simulink model "PassVeh14DOF"  (R2026b)
settings: Solver=ode23tb  StopTime=inf  FixedStep=.001  RelTol=1e-1  EnableMultiTasking=on
model workspace (MAT data in the model file):
  AlgnTrqCambCompl = [0 0 0 0]
  AlgnTrqSteerCompl = [0 0 0 0]
  AxlIxx = 62.3745166667
  AxlM = 160
  BumpCamber = [0 0 0 0]
  BumpCaster = [0 0 0 0]
  BumpSteer = [0 0 0 0]
  CambVsSteerAng = [0 0 0 0]
  CastVsSteerAng = [0 0 0 0]
  Cps = 2
  Cz = 5565.2246438
  CzWhlAxl = 11490.971257
  DCT_Param : object (value not decoded)
  Downshift_Speeds = [9.5625 12.9375 16.3125 19.6875 23.0625 26.4375 29.8125 33.1875 36.5625 39.9375 43.3125 46.6875 ... (28 elements, 4x7)]
  F0z = [2886 2907]
  F0zWhlAxl = 2907
  Hmax = 0.25
  Kz = 52451.0065793
  KzWhlAxl = 138031.612078
  LatCambCompl = [0 0 0 0]
  LatSteerCompl = [0 0 0 0]
  LatWhlCtrComplLat = [0 0 0 0]
  LatWhlCtrComplLng = [0  0  0  0; 0  0  0  0]
  LatWhlCtrDisp = [0 0 0 0]
  LngCambCompl = [0  0  0  0; 0  0  0  0]
  LngCastCompl = [0  0  0  0; 0  0  0  0]
  LngSteerCompl = [0  0  0  0; 0  0  0  0]
  LngWhlCtrCompl = [0  0  0  0; 0  0  0  0]
  LngWhlCtrDisp = [0 0 0 0]
  MotRatios = [1 1]
  NCyl = 6
  NrmlWhlFrcOff = [2886 2886 2907 2907]
  NrmlWhlRates = [52.4510065793 52.4510065793 52.4510065793 52.4510065793]
  Pedal_Positions = [0.1 0.4 0.5 0.9]
  Pstd = 101325
  Rair = 287
  RollCamber : object (value not decoded)
  RollCaster : object (value not decoded)
  RollSteer : object (value not decoded)
  RollStiffArb = [0 0]
  RollStiffArbFrnt = 800
  RollStiffNoArb = [0 0]
  RollStiffNoArbFrnt = 0
  RollStiffNoTwstRear = 0
  ShckFrcVsCompRate = [5.5652246438 5.5652246438 5.5652246438 5.5652246438]
  StatCamber = [0 0 0 0]
  StatCaster = [0 0 0 0]
  StatLdWhlR = [0.3 0.3 0.3 0.3]
  StatToe = [0 0 0 0]
  Trans : object (value not decoded)
  Tstd = 293.15
  Upshift_Speeds = [12.9375 16.3125 19.6875 33 26.4375 29.8125 33.1875 52.5 39.9375 43.3125 46.6875 77.25 ... (28 elements, 4x7)]
  VEH : object (value not decoded)
  Vd = 0.00346
  VrtLdTrnsfr = [0 0 0 0]
  WH : Mass (value not decoded)
  dt3D = 0.05
  f_air = [0 0 0 0 0 0 0 0 0 0 0 0 ... (256 elements, 16x16)]
  f_co = [0 0 0 0 0 0 0 0 0 0 0 0 ... (256 elements, 16x16)]
  f_co2 = [0 0 0 0 0 0 0 0 0 0 0 0 ... (256 elements, 16x16)]
  f_eff = [352.135682859 352.135682859 320.724378192 303.655312657 295.930136708 291.240087194 291.240271258 291.240312459 291.240275452 291.240198499 291.240100781 291.240018769 ... (256 elements, 16x16)]
  f_fuel = [0 0 0 0 0 0 0 0 0 0 0 0 ... (256 elements, 16x16)]
  f_hc = [0 0 0 0 0 0 0 0 0 0 0 0 ... (256 elements, 16x16)]
  f_nox = [0 0 0 0 0 0 0 0 0 0 0 0 ... (256 elements, 16x16)]
  f_pm = [0 0 0 0 0 0 0 0 0 0 0 0 ... (256 elements, 16x16)]
  f_susp_axl_bp = [1 2]
  f_susp_dz_bp = [-0.325022776267 -0.315022776267 -0.305022776267 -0.205022776267 -0.105022776267 -0.00502277626717 0.0949772237328 0.194977223733 0.204977223733 0.214977223733]
  f_susp_dzdot_bp = [-3 -0.3 -0.2 -0.1 0 0.1 0.2 0.3 3]
  f_susp_fmz = [-144070.391448 -93629.24037 -75929.1118915 -20630.5828179 -15385.48216 -10140.3815021 -4895.28084414 349.819813785 -31916.3973792 18437.6709544 -83996.1993354 -33555.0482577 ... (43920 elements, 10x9x61x2x4)]
  f_susp_geom = [0 0 0 0 0 0 0 0 0 0 0 0 ... (3660 elements, 10x61x2x3)]
  f_susp_strgdelta_bp = [-0.523598775598 -0.506145483078 -0.488692190558 -0.471238898038 -0.453785605519 -0.436332312999 -0.418879020479 -0.401425727959 -0.383972435439 -0.366519142919 -0.349065850399 -0.331612557879 ... (61 elements, 1x61)]
  f_tbrake = [0 76.8593923996 105.140482948 131.533638111 157.926793274 176.658631717 176.65727296 176.656856686 176.656879077 176.657093756 176.657404516 176.65772406 ... (256 elements, 16x16)]
  f_tbrake_n_bpt = [0 649.519052838 912.419621844 1175.32019085 1438.22075986 1701.12132886 1964.02189787 2226.92246687 2489.82303588 2752.72360489 3015.62417389 3278.5247429 ... (16 elements, 1x16)]
  f_tbrake_t_bpt = [0 34.6410161514 61.0341713143 87.4273264773 113.82048164 140.213636803 166.606791966 192.999947129 219.393102292 245.786257455 272.179412618 298.572567781 ... (16 elements, 1x16)]
  f_texh = [766.752464599 766.752464599 786.17542386 801.679939032 884.591982581 910.574397722 910.571871054 910.570774534 910.570601632 910.570821151 910.571247242 910.571639815 ... (256 elements, 16x16)]
  f_twc_eff_co = [0.17 0.25 0.45 0.99 0.99 0.99 0.99]
  f_twc_eff_hc = [0.21 0.375 0.75 0.98 0.98 0.98 0.98]
  f_twc_eff_lam = [0.909090909 0.944055944 0.979020979 1 1.013986014 1.048951049 1.083916084]
  f_twc_eff_nox = [0.98 0.98 0.98 0.97 0.05 0.02 0]
  numWheel = 4
symbols that are objects in the model workspace (value not decoded): VEH
libraries: vehdynlibtire x12, vehdynlibsuspension x8, autolibutils x5, sharedtransform x5, shared6dof x2, vehdynlibeom x1, vehdynlibtirecommon x1, matrix_library x1
(part 2 of 9)

== system PassVeh14DOF/Suspension ==
  Steering : Inport
  Vehicle : Inport  Port=2
  Wheel : Inport  Port=3
  Double Wishbone Suspension : Subsystem  VariantControl=1
      mask Display: image('suspdw.png');
  Independent Mapped Front Suspension Mapped Solid Axle Rear Suspension : Subsystem  VariantControl=2
      mask Display: image([imread('suspindmap.png');imread('suspsamap.png')]);
  Kinematics and Compliance Independent Suspension : Subsystem  VariantControl=6
      mask Display: image('suspkandc.png');
  MacPherson Front Suspension Solid Axle Rear Suspension : Subsystem  VariantControl=3
      mask Display: image([imread('suspmacp.png');imread('suspsacoil.png')]);
  MacPherson Suspension : Subsystem  VariantControl=4
      mask Display: image('suspmacp.png');
  Mapped Suspension : Subsystem  VariantControl=5
      mask Display: image('suspindmap.png');
  Suspension : Outport  VectorParamsAs1DForOutWhenUnconnected=off

== system PassVeh14DOF/Vehicle ==
  Suspension : Inport
  Wind : Inport  Port=2
  Constant1 : Constant  Value=[0;0;0]
  Suspension to Chasiss Transforms : Subsystem
  Terminator{,1..5} (6 alike) : Terminator
  Vehicle Body 6DOF : vehdynlibeom/Vehicle Body 6DOF  extPos=on  extVel=on  extEuler=on  extRotRate=on  htchFMode=off  htchMMode=off  m=VEH.Mass  a=VEH.FrontAxlePositionfromCG  b=VEH.RearAxlePositionfromCG  d=0  h=VEH.HeightCG  dh=1  hl=0  hh=0.1  Xe_o=[VEH.InitialLongPosition,VEH.InitialLatPosition,VEH.InitialVertPosition]  xbdot_o=[VEH.InitialLongVel,VEH.InitialLatVel,VEH.InitialVertVel]  eul_o=[VEH.InitialRollAngle,VEH.InitialPitchAngle,VEH.InitialYawAngle]  p_o=[VEH.InitialRollRate,VEH.InitialPitchRate,VEH.InitialYawRate]  Iveh=[VEH.RollMomentInertia 0 0; 0 VEH.PitchMomentInertia 0; 0 0 VEH.YawMomentInertia]  w=VEH.TrackWidth.*[1 1]  z1m=0  z1R=[-.25,.125,.15]  z1I=[1.4,-.2,.1;-.2,1.4,.1;.1,.1,2.25].*0  z2m=0  z2R=[1.4,0,.8]  z2I=[1.4,-.2,.1;-.2,1.4,.1;.1,.1,2.25].*0  z3m=0  z3R=[.75,-.5,.4]  z3I=[5,-.1,-2;-2,9,.1;-.1,.1,6].*0  z4m=0  z4R=[.75,.5,.4]  z4I=[5,-.1,-2;-2,9,.1;-.1,.1,6].*0  z5m=0  z5R=[1.25,-.5,.4]  z5I=[5,-.1,-2;-2,9,.1;-.1,.1,6].*0  z6m=0  z6R=[1.25,-.5,.4]  z6I=[5,-.1,-2;-2,9,.1;-.1,.1,6].*0  z7m=0  z7R=[2,0,.25]  z7I=[1.4,-.2,.1;-.2,1.4,.1;.1,.1,2.25].*0  Af=VEH.FrontalArea  Cd=.3  Cl=.1  Cpm=.1  beta_w=[0,0.1745,0.3491,0.5236,0.6981,0.8727,1.0472,1.2217,1.3963,1.5708]  Cs=[0.1000,0.1000,0.1000,0.1000,0.1000,0.1000,0.1000,0.1000,0.1000,0.1000]  Cym=[0,0,0.0667,0.1000,0.1333,0.1667,0.2000,0.2333,0.2667,0.3000]  Pabs=101325  extTamb=off  Tair=273  g=9.81  xdot_tol=.1  longOff=0  latOff=0  vertOff=0.0112  wrapAng=off  aMode=2
  VehFdbk : Outport  VectorParamsAs1DForOutWhenUnconnected=off
  wires:
  Vehicle Body 6DOF/1 -> VehFdbk/1, Suspension to Chasiss Transforms/1(VehFdbk)  "VehFdbk"
  Vehicle Body 6DOF/7 -> Terminator5/1
  Constant1/1 -> Vehicle Body 6DOF/4
  Wind/1 -> Vehicle Body 6DOF/5
  Vehicle Body 6DOF/2 -> Terminator/1
  Suspension/1 -> Suspension to Chasiss Transforms/2(Suspension)
  Suspension to Chasiss Transforms/1(FsB) -> Vehicle Body 6DOF/1
  Suspension to Chasiss Transforms/3(Fext) -> Vehicle Body 6DOF/3
  Vehicle Body 6DOF/5 -> Terminator3/1
  Vehicle Body 6DOF/6 -> Terminator4/1
  Vehicle Body 6DOF/3 -> Terminator1/1
  Vehicle Body 6DOF/4 -> Terminator2/1
  Suspension to Chasiss Transforms/2(MsB) -> Vehicle Body 6DOF/2

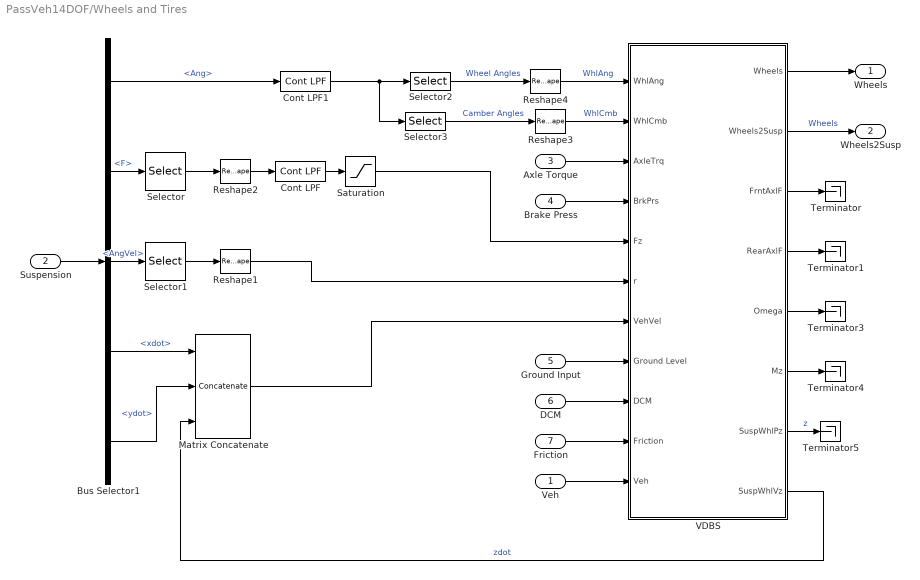
== system PassVeh14DOF/Wheels and Tires ==
  Veh : Inport
  Suspension : Inport  Port=2
  Axle Torque : Inport  Port=3
  Brake Press : Inport  Port=4  Unit=Pa
  Ground Input : Inport  Port=5
  DCM : Inport  Port=6
  Friction : Inport  Port=7  PortDimensions=4
  Bus Selector1 : BusSelector  OutputSignals=Whl.Ang,Whl.F,Whl.AngVel,Whl.xdot,Whl.ydot
  Cont LPF : autolibutils/Cont LPF  wc=100*2*pi  AbsoluteTolerance=auto  aMode=2
  Cont LPF1 : autolibutils/Cont LPF  wc=100*2*pi  AbsoluteTolerance=1e-2  aMode=2
  Matrix Concatenate : Concatenate  NumInputs=3  Mode=Multidimensional array
  Reshape{1..4} (4 alike) : Reshape
  Saturation : Saturate  UpperLimit=inf  LowerLimit=-10*9.81*2000  ZeroCross=off
  Selector : Selector  NumberOfDimensions=2  InputPortWidth=3  IndexOptions=Index vector (dialog),Select all  Indices=[3],1  OutputSizes=1,1
  Selector1 : Selector  NumberOfDimensions=2  InputPortWidth=1  IndexOptions=Index vector (dialog),Select all  Indices=[3],1  OutputSizes=1,1
  Selector2 : Selector  NumberOfDimensions=2  InputPortWidth=3  IndexOptions=Index vector (dialog),Select all  Indices=3,1  OutputSizes=1,1
  Selector3 : Selector  NumberOfDimensions=2  InputPortWidth=3  IndexOptions=Index vector (dialog),Select all  Indices=1,1  OutputSizes=1,1
  Terminator{,1,3..5} (5 alike) : Terminator
  VDBS : Subsystem  VariantControl=0
  Wheels : Outport  VectorParamsAs1DForOutWhenUnconnected=off
  Wheels2Susp : Outport  Port=2  VectorParamsAs1DForOutWhenUnconnected=off
  wires:
  Bus Selector1/2 -> Selector/1  "<F>"
  VDBS/3(FrntAxlF) -> Terminator/1
  VDBS/4(RearAxlF) -> Terminator1/1
  VDBS/5(Omega) -> Terminator3/1
  VDBS/6(Mz) -> Terminator4/1
  Selector1/1 -> Reshape1/1
  Matrix Concatenate/1 -> VDBS/7(VehVel)
  Axle Torque/1 -> VDBS/3(AxleTrq)
  Reshape4/1 -> VDBS/1(WhlAng)  "WhlAng"
  Reshape3/1 -> VDBS/2(WhlCmb)  "WhlCmb"
  Selector/1 -> Reshape2/1
  Saturation/1 -> VDBS/5(Fz)
  Ground Input/1 -> VDBS/8(Ground Level)
  VDBS/8(SuspWhlVz) -> Matrix Concatenate/3  "zdot"
  Bus Selector1/1 -> Cont LPF1/1  "<Ang>"
  Selector3/1 -> Reshape3/1  "Camber Angles"
  Suspension/1 -> Bus Selector1/1
  Bus Selector1/4 -> Matrix Concatenate/1  "<xdot>"
  Bus Selector1/5 -> Matrix Concatenate/2  "<ydot>"
  VDBS/7(SuspWhlPz) -> Terminator5/1  "z"
  Reshape2/1 -> Cont LPF/1
  Bus Selector1/3 -> Selector1/1  "<AngVel>"
  Reshape1/1 -> VDBS/6(r)
  Brake Press/1 -> VDBS/4(BrkPrs)
  Friction/1 -> VDBS/10(Friction)
  Cont LPF/1 -> Saturation/1
  Cont LPF1/1 -> Selector3/1, Selector2/1
  Selector2/1 -> Reshape4/1  "Wheel Angles"
  Veh/1 -> VDBS/11(Veh)
  VDBS/2(Wheels2Susp) -> Wheels2Susp/1  "Wheels"
  VDBS/1(Wheels) -> Wheels/1
  DCM/1 -> VDBS/9(DCM)

== system PassVeh14DOF/Suspension/Double Wishbone Suspension ==
  Wheel : Inport
  Steering : Inport  Port=2
  Vehicle : Inport  Port=3
  Bus Creator1 : BusCreator  Inputs=6
  Bus Creator2 : BusCreator  Inputs=2
  Bus Creator3 : BusCreator  Inputs=2
  Bus Creator4 : BusCreator  Inputs=6
  Bus Selector : BusSelector  OutputSignals=z,RL,zdot,Fx,Fy,M
  Bus Selector1 : BusSelector  OutputSignals=P,V
  Bus Selector2 : BusSelector  OutputSignals=SuspFrame.z
  Independent Suspension – Double Wishbone : vehdynlibsuspension/Independent Suspension - Double Wishbone  ActiveDampEn=off  NumAxl=2  NumWhlsByAxl=[2 2]  StrgEnByAxl=[1 0]  AntiSwayEnByAxl=[1 0]  WhlNumVec="[1  2  1  2]"  AxleNumVec="[1  1  2  2]"  SuspTypesByAxle="[1  1]"  SuspImage=suspdw.png  IdealSuspEn=on  IdealSuspAxles="[1  2]"  Kz=Kz  F0z=F0z  Cz=Cz  Hmax=Hmax  f_act_susp_cz=[10000 10000;10000 10000]  f_act_susp_duty_bpt=[0 1]  f_act_susp_zdot_bpt=[-1 1]  Toe=0.  RollStrgSlp=0.  ToeStrgSlp=0.  Caster=0.  CasterHslp=0.  CasterStrgSlp=0.  Camber=0.  CamberHslp=0.  CamberStrgSlp=0.  StrgHgtSlp=0.1432  MappedSuspEn=off  MappedSuspAxles="[1  2]"  f_susp_axl_bp=[1 2]  f_susp_dz_bp=[-0.15 -0.14 -0.13 -0.12 -0.11 -0.10 -0.09 -0.08 -0.07 -0.06 -0.05 -0.04 -0.03 -0.02 -0.01 0.00 0.01 0.02 0.03 0.04 0.05 0.06 0.07 0.08 0.09 0.10 0.11 0.12 0.13 0.14 0.15]  f_susp_dzdot_bp=[-0.15 -0.14 -0.13 -0.12 -0.11 -0.10 -0.09 -0.08 -0.07 -0.06 -0.05 -0.04 -0.03 -0.02 -0.01 0.00 0.01 0.02 0.03 0.04 0.05 0.06 0.07 0.08 0.09 0.10 0.11 0.12 0.13 0.14 0.15]  f_susp_fmz=zeros(31,31,61,2,4)  f_susp_geom=zeros(31,61,2,3)  f_susp_strgdelta_bp=[-30,-29,-28,-27,-26,-25,-24,-23,-22,-21,-20,-19,-18,-17,-16,-15,-14,-13,-12,-11,-10,-9,-8,-7,-6,-5,-4,-3,-2,-1,0,1,2,3,4,5,6,7,8,9,10,11,12,13,14,15,16,17,18,19,20,21,22,23,24,25,26,27,28,29,30]  AntiSwayR=0.2  AntiSwayNtrlAng=0.5236  AntiSwayTrsK=8e2
  Selector1 : Selector  NumberOfDimensions=2  IndexOptions=Index vector (dialog),Select all  Indices=1,1  OutputSizes=1,1
  Selector2 : Selector  NumberOfDimensions=2  IndexOptions=Index vector (dialog),Select all  Indices=2,1  OutputSizes=1,1
  Steer Rate Adapter : Subsystem
  Steering Adapter : Subsystem
  Terminator : Terminator
  Terminator1 : Terminator
  Vehicle Adapter : Subsystem
  Wheel  Adapter : Subsystem
  Wheel1 : InportShadow
  Suspension : Outport  VectorParamsAs1DForOutWhenUnconnected=off
  wires:
  Bus Creator3/1 -> Suspension/1
  Steering Adapter/1(StrgAng) -> Independent Suspension – Double Wishbone/9
  Independent Suspension – Double Wishbone/1 -> Terminator/1
  Wheel  Adapter/6(RL) -> Bus Creator4/6
  Bus Selector1/1 -> Independent Suspension – Double Wishbone/7  "<P>"
  Wheel  Adapter/2(WhlFy) -> Bus Creator4/2  "Fy"
  Wheel/1 -> Wheel  Adapter/1(Wheels)
  Steer Rate Adapter/1(AngVel) -> Bus Creator1/6  "AngVel"
  Bus Creator4/1 -> Bus Selector/1
  Bus Creator2/1 -> Bus Creator3/1  "Veh"
  Vehicle Adapter/2(VehVbody) -> Selector1/1, Selector2/1  "V"
  Selector2/1 -> Bus Creator1/3  "ydot"
  Bus Selector1/2 -> Independent Suspension – Double Wishbone/8  "<V>"
  Independent Suspension – Double Wishbone/2 -> Bus Creator2/1  "F"
  Bus Selector/2 -> Independent Suspension – Double Wishbone/2  "<RL>"
  Wheel  Adapter/5(M) -> Bus Creator4/5  "M"
  Bus Selector/4 -> Independent Suspension – Double Wishbone/4  "<Fx>"
  Independent Suspension – Double Wishbone/4 -> Bus Creator1/1  "F"
  Steering/1 -> Steering Adapter/1(Steer)
  Selector1/1 -> Bus Creator1/2  "xdot"
  Independent Suspension – Double Wishbone/3 -> Bus Creator2/2  "M"
  Vehicle Adapter/1(VehSusp) -> Bus Selector1/1
  Wheel  Adapter/4(zdot) -> Bus Creator4/4
  Vehicle/1 -> Vehicle Adapter/1(Veh), Steer Rate Adapter/1(Veh)
  Bus Selector/6 -> Independent Suspension – Double Wishbone/6  "<M>"
  Bus Selector/5 -> Independent Suspension – Double Wishbone/5  "<Fy>"
  Bus Selector/1 -> Independent Suspension – Double Wishbone/1  "<z>"
  Wheel  Adapter/3(z) -> Bus Creator4/3
  Independent Suspension – Double Wishbone/6 -> Bus Creator1/4  "Ang"
  Bus Creator1/1 -> Bus Creator3/2  "Whl"
  Wheel  Adapter/1(WhlFx) -> Bus Creator4/1  "Fx"
  Bus Selector/3 -> Independent Suspension – Double Wishbone/3  "<zdot>"
  Independent Suspension – Double Wishbone/5 -> Terminator1/1  "V"
  Bus Selector2/1 -> Bus Creator1/5  "<z>"
  Wheel1/1 -> Bus Selector2/1

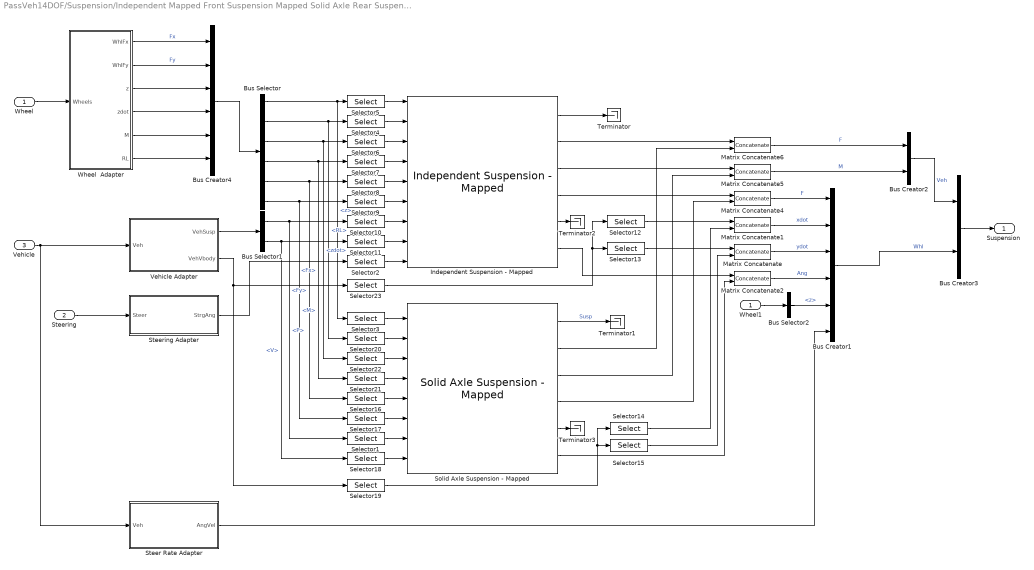
== system PassVeh14DOF/Suspension/Independent Mapped Front Suspension Mapped Solid Axle Rear Suspension ==
  Wheel : Inport
  Steering : Inport  Port=2
  Vehicle : Inport  Port=3
  Bus Creator1 : BusCreator  Inputs=6
  Bus Creator2 : BusCreator  Inputs=2
  Bus Creator3 : BusCreator  Inputs=2
  Bus Creator4 : BusCreator  Inputs=6
  Bus Selector : BusSelector  OutputSignals=z,RL,zdot,Fx,Fy,M
  Bus Selector1 : BusSelector  OutputSignals=P,V
  Bus Selector2 : BusSelector  OutputSignals=SuspFrame.z
  Independent Suspension - Mapped : vehdynlibsuspension/Independent Suspension - Mapped  NumAxl=1  NumWhlsByAxl=2  StrgEnByAxl=1  AntiSwayEnByAxl=1  WhlNumVec="[1  2]"  AxleNumVec="[1  1]"  SuspTypesByAxle=[2]  SuspImage=suspindmap.png  IdealSuspEn=off  IdealSuspAxles="[1  2]"  Kz=64370  F0z=9810  Cz=10000  Hmax=0.5  Toe=2  RollStrgSlp=-13  ToeStrgSlp=0.01  Caster=4  CasterHslp=-13  CasterStrgSlp=0.01  Camber=4  CamberHslp=-13  CamberStrgSlp=0.01  StrgHgtSlp=0.0025  MappedSuspEn=on  MappedSuspAxles=[1]  f_susp_axl_bp=[1 2]  f_susp_dz_bp=f_susp_dz_bp  f_susp_dzdot_bp=f_susp_dzdot_bp  f_susp_fmz=f_susp_fmz  f_susp_geom=f_susp_geom  f_susp_strgdelta_bp=f_susp_strgdelta_bp  NDFLookupOutType=1:4  NDGLookupOutType=1:3  AntiSwayR=0.2  AntiSwayNtrlAng=0.5236  AntiSwayTrsK=8e2
  Matrix Concatenate{,1..2,4..6} (6 alike) : Concatenate  Mode=Multidimensional array  ConcatenateDimension=2
  Selector{1,17..19} (4 alike) : Selector  NumberOfDimensions=2  IndexOptions=Select all,Index vector (dialog)  Indices=[1 2],[3 4]  OutputSizes=1,1
  Selector{9..11,23} (4 alike) : Selector  NumberOfDimensions=2  IndexOptions=Select all,Index vector (dialog)  Indices=[1 2],[1 2]  OutputSizes=1,1
  Selector12 : Selector  NumberOfDimensions=2  InputPortWidth=3  IndexOptions=Index vector (dialog),Select all  Indices=1,1  OutputSizes=1,1
  Selector13 : Selector  NumberOfDimensions=2  InputPortWidth=3  IndexOptions=Index vector (dialog),Select all  Indices=2,1  OutputSizes=1,1
  Selector14 : Selector  NumberOfDimensions=2  InputPortWidth=3  IndexOptions=Index vector (dialog),Select all  Indices=1,1  OutputSizes=1,1
  Selector15 : Selector  NumberOfDimensions=2  InputPortWidth=3  IndexOptions=Index vector (dialog),Select all  Indices=2,1  OutputSizes=1,1
  Selector{3,16,20..22} (5 alike) : Selector  IndexOptions=Index vector (dialog)  Indices=[3 4]  OutputSizes=1
  Selector{2,4..8} (6 alike) : Selector  IndexOptions=Index vector (dialog)  Indices=[1 2]  OutputSizes=1
  Solid Axle Suspension - Mapped : vehdynlibsuspension/Solid Axle Suspension - Mapped  NumAxl=1  NumWhlsByAxl=2  StrgEnByAxl=0  WhlNumVec="[1  2]"  AxleNumVec="[1  1]"  SuspTypesByAxle=[2]  SuspImage=suspsamap.png  AxlIxx=AxlIxx  AxlM=AxlM  TrackCoords=[0 0;VEH.TrackWidth*[-1 1]/2;0 0]  SuspCoords=[0 0;VEH.TrackWidth*[-1 1]/2;0 0]  KzWhlAxl=KzWhlAxl  F0zWhlAxl=F0zWhlAxl  CzWhlAxl=CzWhlAxl  IdealSuspEn=off  IdealSuspAxles="[1  2]"  Kz=64370  F0z=9810  Cz=10000  Hmax=0.5  Toe=2  RollStrgSlp=-13  ToeStrgSlp=0.01  Caster=4  CasterHslp=-13  CasterStrgSlp=0.01  Camber=4  CamberHslp=-13  CamberStrgSlp=0.01  StrgHgtSlp=0.0025  MappedSuspEn=on  MappedSuspAxles=[1]  f_susp_axl_bp=[1 2]  f_susp_dz_bp=f_susp_dz_bp  f_susp_dzdot_bp=f_susp_dzdot_bp  f_susp_fmz=f_susp_fmz  f_susp_geom=f_susp_geom  f_susp_strgdelta_bp=f_susp_strgdelta_bp  NDFLookupOutType=1:4  NDGLookupOutType=1:3
  Steer Rate Adapter : Subsystem
  Steering Adapter : Subsystem
  Terminator{,1..3} (4 alike) : Terminator
  Vehicle Adapter : Subsystem
  Wheel  Adapter : Subsystem
  Wheel1 : InportShadow
  Suspension : Outport  VectorParamsAs1DForOutWhenUnconnected=off
  wires:
  Vehicle Adapter/2(VehVbody) -> Selector19/1, Selector23/1
  Selector22/1 -> Solid Axle Suspension - Mapped/3
  Bus Selector/3 -> Selector22/1, Selector6/1  "<zdot>"
  Solid Axle Suspension - Mapped/4 -> Matrix Concatenate4/2
  Solid Axle Suspension - Mapped/1 -> Terminator1/1  "Susp"
  Selector12/1 -> Matrix Concatenate1/1
  Selector7/1 -> Independent Suspension - Mapped/4
  Selector18/1 -> Solid Axle Suspension - Mapped/8
  Selector13/1 -> Matrix Concatenate/1
  Selector14/1 -> Matrix Concatenate1/2
  Selector21/1 -> Solid Axle Suspension - Mapped/4
  Vehicle/1 -> Vehicle Adapter/1(Veh), Steer Rate Adapter/1(Veh)
  Wheel  Adapter/4(zdot) -> Bus Creator4/4
  Solid Axle Suspension - Mapped/3 -> Matrix Concatenate5/2
  Selector1/1 -> Solid Axle Suspension - Mapped/7
  Matrix Concatenate4/1 -> Bus Creator1/1  "F"
  Selector16/1 -> Solid Axle Suspension - Mapped/5
  Matrix Concatenate5/1 -> Bus Creator2/2  "M"
  Independent Suspension - Mapped/4 -> Matrix Concatenate4/1
  Selector4/1 -> Independent Suspension - Mapped/2
  Selector10/1 -> Independent Suspension - Mapped/7
  Selector9/1 -> Independent Suspension - Mapped/6
  Wheel  Adapter/3(z) -> Bus Creator4/3
  Solid Axle Suspension - Mapped/2 -> Matrix Concatenate6/2
  Wheel/1 -> Wheel  Adapter/1(Wheels)
  Selector5/1 -> Independent Suspension - Mapped/1
  Independent Suspension - Mapped/3 -> Matrix Concatenate5/1
  Selector8/1 -> Independent Suspension - Mapped/5
  Independent Suspension - Mapped/2 -> Matrix Concatenate6/1
  Independent Suspension - Mapped/6 -> Matrix Concatenate2/1
  Selector20/1 -> Solid Axle Suspension - Mapped/2
  Independent Suspension - Mapped/1 -> Terminator/1
  Bus Creator2/1 -> Bus Creator3/1  "Veh"
  Bus Selector/4 -> Selector7/1, Selector21/1  "<Fx>"
  Matrix Concatenate2/1 -> Bus Creator1/4  "Ang"
  Wheel  Adapter/2(WhlFy) -> Bus Creator4/2  "Fy"
  Bus Creator4/1 -> Bus Selector/1
  Selector17/1 -> Solid Axle Suspension - Mapped/6
  Selector2/1 -> Independent Suspension - Mapped/9
  Wheel  Adapter/5(M) -> Bus Creator4/5
  Matrix Concatenate/1 -> Bus Creator1/3  "ydot"
  Steering/1 -> Steering Adapter/1(Steer)
  Matrix Concatenate1/1 -> Bus Creator1/2  "xdot"
  Selector15/1 -> Matrix Concatenate/2
  Selector3/1 -> Solid Axle Suspension - Mapped/1
  Bus Selector1/2 -> Selector11/1, Selector18/1  "<V>"
  Vehicle Adapter/1(VehSusp) -> Bus Selector1/1
  Steering Adapter/1(StrgAng) -> Selector2/1
  Selector6/1 -> Independent Suspension - Mapped/3
  Bus Selector/6 -> Selector9/1, Selector17/1  "<M>"
  Wheel  Adapter/1(WhlFx) -> Bus Creator4/1  "Fx"
  Selector11/1 -> Independent Suspension - Mapped/8
  Wheel  Adapter/6(RL) -> Bus Creator4/6
  Matrix Concatenate6/1 -> Bus Creator2/1  "F"
  Bus Selector1/1 -> Selector10/1, Selector1/1  "<P>"
  Solid Axle Suspension - Mapped/6 -> Matrix Concatenate2/2
  Bus Selector/1 -> Selector3/1, Selector5/1  "<z>"
  Bus Selector/5 -> Selector8/1, Selector16/1  "<Fy>"
  Bus Creator1/1 -> Bus Creator3/2  "Whl"
  Bus Creator3/1 -> Suspension/1
  Bus Selector/2 -> Selector20/1, Selector4/1  "<RL>"
  Steer Rate Adapter/1(AngVel) -> Bus Creator1/6
  Independent Suspension - Mapped/5 -> Terminator2/1
  Solid Axle Suspension - Mapped/5 -> Terminator3/1
  Selector19/1 -> Selector14/1, Selector15/1
  Selector23/1 -> Selector12/1, Selector13/1
  Bus Selector2/1 -> Bus Creator1/5  "<z>"
  Wheel1/1 -> Bus Selector2/1

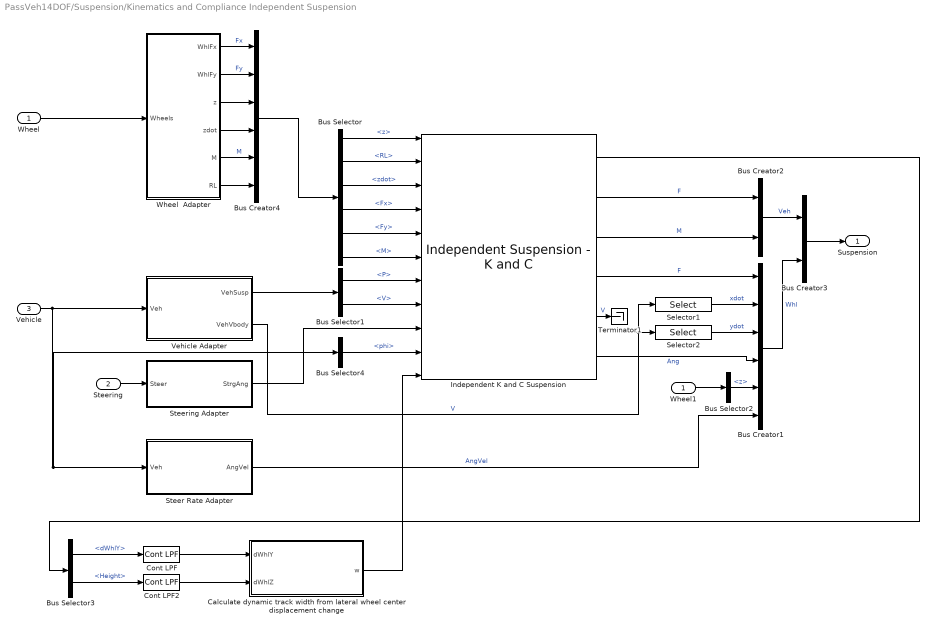
== system PassVeh14DOF/Suspension/Kinematics and Compliance Independent Suspension ==
  Wheel : Inport
  Steering : Inport  Port=2
  Vehicle : Inport  Port=3
  Bus Creator1 : BusCreator  Inputs=6
  Bus Creator2 : BusCreator  Inputs=2
  Bus Creator3 : BusCreator  Inputs=2
  Bus Creator4 : BusCreator  Inputs=6
  Bus Selector : BusSelector  OutputSignals=z,RL,zdot,Fx,Fy,M
  Bus Selector1 : BusSelector  OutputSignals=P,V
  Bus Selector2 : BusSelector  OutputSignals=SuspFrame.z
  Bus Selector3 : BusSelector  OutputSignals=dWhlY,Height
  Bus Selector4 : BusSelector  OutputSignals=InertFrm.Cg.Ang.phi
  Calculate dynamic track width from lateral wheel center displacement change : Subsystem  mask{w=VEH.TrackWidth.*[1 1]}
      mask prompts: w "vdynblks:vehdynVehBody6Dof:blkPrm_w"
      mask DialogControl w Prompt: Track widths [front, rear], w [m]:
  Cont LPF : autolibutils/Cont LPF  wc=100*2*pi  AbsoluteTolerance=auto  aMode=2
  Cont LPF2 : autolibutils/Cont LPF  wc=100*2*pi  AbsoluteTolerance=auto  aMode=2
  Independent K and C Suspension : vehdynlibsuspension/Independent Suspension - K and C  ActiveDampEn=off  NumAxl=2  NumWhlsByAxl=[2 2]  StrgEnByAxl=[1 0]  AntiSwayEnByAxl=[0 0]  WhlNumVec="[1  2  1  2]"  AxleNumVec="[1  1  2  2]"  SuspTypesByAxle="[1  1]"  SuspImage=suspkandc.png  IdealSuspEn=on  IdealSuspAxles="[1  2]"  tanTheta_FL=[0 0 0]  tanTheta_FR=[0 0 0]  tanTheta_RL=[0 0 0]  tanTheta_RR=[0 0 0]  SteerSign=1  LongitudinalSign=1  LateralSign=1  VerticalSign=1  WhlMzSign=1  tanTheta_SVSA_WC_FL=1  tanTheta_SVSA_WC_FR=1  tanTheta_SVSA_WC_RL=1  tanTheta_SVSA_WC_RR=1  tanTheta_SVSA_CP_FL=1  tanTheta_SVSA_CP_FR=1  tanTheta_SVSA_CP_RL=1  tanTheta_SVSA_CP_RR=1  SuspType=Independent front and rear  DrivetrainType=FWD  StrPlusDirection=Right  XPlusDirection=Front  YPlusDirection=Right  ZPlusDirection=Up  WhlMzDirection=Counter-clockwise  ShockType=Constant  ShckFrcVsCompRate=ShckFrcVsCompRate  MotRatios=MotRatios  BumpSteer=BumpSteer  BumpCamber=BumpCamber  BumpCaster=BumpCaster  LatWhlCtrDisp=LatWhlCtrDisp  LngWhlCtrDisp=LngWhlCtrDisp  NrmlWhlRates=NrmlWhlRates  NrmlWhlFrcOff=NrmlWhlFrcOff  RollSteer=RollSteer  RollCamber=RollCamber  RollCaster=RollCaster  RollStiffArb=RollStiffArb  RollStiffNoArb=RollStiffNoArb  RollStiffArbFrnt=RollStiffArbFrnt  RollStiffNoArbFrnt=RollStiffNoArbFrnt  RollStiffNoTwstRear=RollStiffNoTwstRear  CambVsSteerAng=CambVsSteerAng  CastVsSteerAng=CastVsSteerAng  LngSteerCompl=LngSteerCompl  LngCambCompl=LngCambCompl  LngCastCompl=LngCastCompl  LngWhlCtrCompl=LngWhlCtrCompl  LatWhlCtrComplLng=LatWhlCtrComplLng  LatSteerCompl=LatSteerCompl  LatCambCompl=LatCambCompl  LatWhlCtrComplLat=LatWhlCtrComplLat  LatSteerComplOpp=struct('FL',[-2. -1.;0 0;2. 1.],'FR',[-2. 1.;0 0;2. -1.],'RL',[-2. -1.;0 0;2. 1.],'RR',[-2. 1.;0 0;2. -1.])  LatCambComplOpp=struct('FL',[-2. -1.;0 0;2. 1.],'FR',[-2. 1.;0 0;2. -1.],'RL',[-2. -1.;0 0;2. 1.],'RR',[-2. 1.;0 0;2. -1.])  LatWhlCtrComplLatOpp=struct('FL',[-2. -5.;0 0;2. 5.],'FR',[-2. 5.;0 0;2. -5.],'RL',[-2. -5.;0 0;2. 5.],'RR',[-2. 5.;0 0;2. -5.])  AlgnTrqSteerCompl=AlgnTrqSteerCompl  AlgnTrqCambCompl=AlgnTrqCambCompl  VrtLdTrnsfr=VrtLdTrnsfr  LatSteerComplPar=struct('FL',[-2. -1.;0 0;2. 1.],'FR',[-2. 1.;0 0;2. -1.],'RL',[-2. -1.;0 0;2. 1.],'RR',[-2. 1.;0 0;2. -1.])  LatCambComplPar=struct('FL',[-2. -1.;0 0;2. 1.],'FR',[-2. 1.;0 0;2. -1.],'RL',[-2. -1.;0 0;2. 1.],'RR',[-2. 1.;0 0;2. -1.])  LatWhlCtrComplLatPar=struct('FL',[-2. -5.;0 0;2. 5.],'FR',[-2. 5.;0 0;2. -5.],'RL',[-2. -5.;0 0;2. 5.],'RR',[-2. 5.;0 0;2. -5.])  StatToe=StatToe  StatCamber=StatCamber  StatCaster=StatCaster  StatLdWhlR=StatLdWhlR  MappedSuspEn=off  RollParamEn=off
  Selector1 : Selector  NumberOfDimensions=2  IndexOptions=Index vector (dialog),Select all  Indices=1,1  OutputSizes=1,1
  Selector2 : Selector  NumberOfDimensions=2  IndexOptions=Index vector (dialog),Select all  Indices=2,1  OutputSizes=1,1
  Steer Rate Adapter : Subsystem
  Steering Adapter : Subsystem
  Terminator1 : Terminator
  Vehicle Adapter : Subsystem
  Wheel  Adapter : Subsystem
  Wheel1 : InportShadow
  Suspension : Outport  VectorParamsAs1DForOutWhenUnconnected=off
  wires:
  Bus Creator3/1 -> Suspension/1
  Bus Creator1/1 -> Bus Creator3/2  "Whl"
  Bus Selector1/2 -> Independent K and C Suspension/8  "<V>"
  Bus Selector/6 -> Independent K and C Suspension/6  "<M>"
  Bus Selector/5 -> Independent K and C Suspension/5  "<Fy>"
  Steering/1 -> Steering Adapter/1(Steer)
  Bus Selector/3 -> Independent K and C Suspension/3  "<zdot>"
  Bus Selector/4 -> Independent K and C Suspension/4  "<Fx>"
  Vehicle/1 -> Vehicle Adapter/1(Veh), Bus Selector4/1, Steer Rate Adapter/1(Veh)
  Vehicle Adapter/1(VehSusp) -> Bus Selector1/1
  Independent K and C Suspension/3 -> Bus Creator2/2  "M"
  Wheel  Adapter/2(WhlFy) -> Bus Creator4/2  "Fy"
  Wheel  Adapter/1(WhlFx) -> Bus Creator4/1  "Fx"
  Wheel/1 -> Wheel  Adapter/1(Wheels)
  Wheel  Adapter/3(z) -> Bus Creator4/3
  Wheel  Adapter/4(zdot) -> Bus Creator4/4
  Wheel  Adapter/5(M) -> Bus Creator4/5  "M"
  Wheel  Adapter/6(RL) -> Bus Creator4/6
  Bus Selector/2 -> Independent K and C Suspension/2  "<RL>"
  Selector1/1 -> Bus Creator1/2  "xdot"
  Selector2/1 -> Bus Creator1/3  "ydot"
  Bus Selector1/1 -> Independent K and C Suspension/7  "<P>"
  Bus Selector/1 -> Independent K and C Suspension/1  "<z>"
  Independent K and C Suspension/4 -> Bus Creator1/1  "F"
  Independent K and C Suspension/6 -> Bus Creator1/4  "Ang"
  Vehicle Adapter/2(VehVbody) -> Selector1/1, Selector2/1  "V"
  Independent K and C Suspension/2 -> Bus Creator2/1  "F"
  Bus Creator2/1 -> Bus Creator3/1  "Veh"
  Bus Creator4/1 -> Bus Selector/1
  Steer Rate Adapter/1(AngVel) -> Bus Creator1/6  "AngVel"
  Steering Adapter/1(StrgAng) -> Independent K and C Suspension/9
  Independent K and C Suspension/1 -> Bus Selector3/1
  Independent K and C Suspension/5 -> Terminator1/1  "V"
  Bus Selector2/1 -> Bus Creator1/5  "<z>"
  Wheel1/1 -> Bus Selector2/1
  Bus Selector4/1 -> Independent K and C Suspension/10  "<phi>"
  Calculate dynamic track width from lateral wheel center displacement change/1(w) -> Independent K and C Suspension/11
  Bus Selector3/1 -> Cont LPF/1  "<dWhlY>"
  Bus Selector3/2 -> Cont LPF2/1  "<Height>"
  Cont LPF/1 -> Calculate dynamic track width from lateral wheel center displacement change/1(dWhlY)
  Cont LPF2/1 -> Calculate dynamic track width from lateral wheel center displacement change/2(dWhlZ)

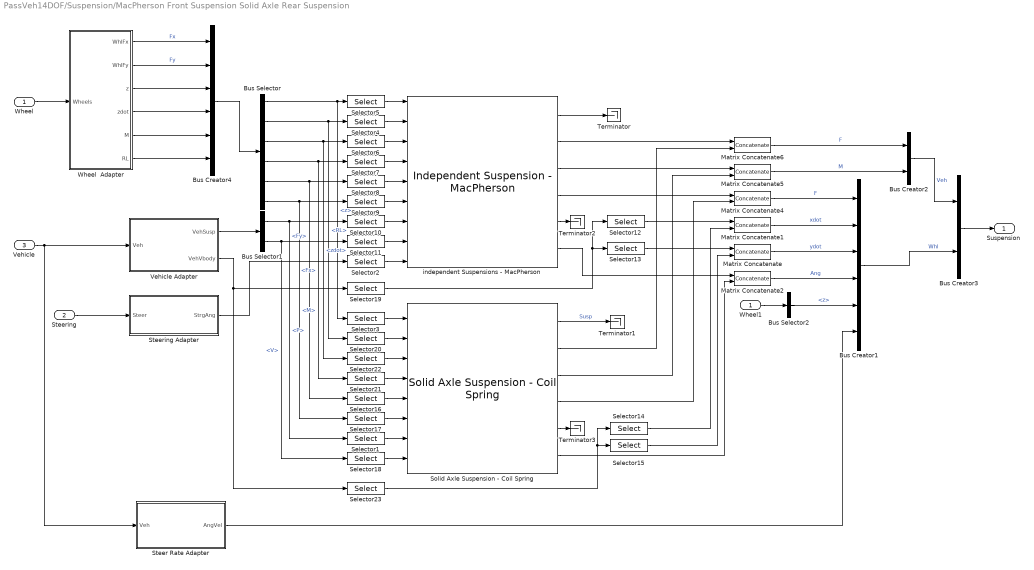
== system PassVeh14DOF/Suspension/MacPherson Front Suspension Solid Axle Rear Suspension ==
  Wheel : Inport
  Steering : Inport  Port=2
  Vehicle : Inport  Port=3
  Bus Creator1 : BusCreator  Inputs=6
  Bus Creator2 : BusCreator  Inputs=2
  Bus Creator3 : BusCreator  Inputs=2
  Bus Creator4 : BusCreator  Inputs=6
  Bus Selector : BusSelector  OutputSignals=z,RL,zdot,Fx,Fy,M
  Bus Selector1 : BusSelector  OutputSignals=P,V
  Bus Selector2 : BusSelector  OutputSignals=SuspFrame.z
  Matrix Concatenate{,1..2,4..6} (6 alike) : Concatenate  Mode=Multidimensional array  ConcatenateDimension=2
  Selector{1,17..18,23} (4 alike) : Selector  NumberOfDimensions=2  IndexOptions=Select all,Index vector (dialog)  Indices=[1 2],[3 4]  OutputSizes=1,1
  Selector{9..11,19} (4 alike) : Selector  NumberOfDimensions=2  IndexOptions=Select all,Index vector (dialog)  Indices=[1 2],[1 2]  OutputSizes=1,1
  Selector12 : Selector  NumberOfDimensions=2  InputPortWidth=3  IndexOptions=Index vector (dialog),Select all  Indices=1,1  OutputSizes=1,1
  Selector13 : Selector  NumberOfDimensions=2  InputPortWidth=3  IndexOptions=Index vector (dialog),Select all  Indices=2,1  OutputSizes=1,1
  Selector14 : Selector  NumberOfDimensions=2  InputPortWidth=3  IndexOptions=Index vector (dialog),Select all  Indices=1,1  OutputSizes=1,1
  Selector15 : Selector  NumberOfDimensions=2  InputPortWidth=3  IndexOptions=Index vector (dialog),Select all  Indices=2,1  OutputSizes=1,1
  Selector{3,16,20..22} (5 alike) : Selector  IndexOptions=Index vector (dialog)  Indices=[3 4]  OutputSizes=1
  Selector{2,4..8} (6 alike) : Selector  IndexOptions=Index vector (dialog)  Indices=[1 2]  OutputSizes=1
  Solid Axle Suspension - Coil Spring : vehdynlibsuspension/Solid Axle Suspension - Coil Spring  NumAxl=1  NumWhlsByAxl=2  StrgEnByAxl=0  WhlNumVec="[1  2]"  AxleNumVec="[1  1]"  SuspTypesByAxle=[1]  SuspImage=suspsacoil.png  AxlIxx=AxlIxx  AxlM=AxlM  TrackCoords=[0 0;VEH.TrackWidth*[-1 1]/2;0 0]  SuspCoords=[0 0;VEH.TrackWidth*[-1 1]/2;0 0]  KzWhlAxl=KzWhlAxl  F0zWhlAxl=F0zWhlAxl  CzWhlAxl=CzWhlAxl  IdealSuspEn=on  IdealSuspAxles=[1]  Kz=Kz  F0z=F0z(2)  Cz=Cz  Hmax=Hmax  Toe=0.  RollStrgSlp=0.  ToeStrgSlp=0  Caster=0.  CasterHslp=0.  CasterStrgSlp=0.01  Camber=0.  CamberHslp=0.  CamberStrgSlp=0.01  StrgHgtSlp=0.1432  MappedSuspEn=off  MappedSuspAxles="[1  2]"  f_susp_axl_bp=[1 2]  f_susp_dz_bp=[-0.15 -0.14 -0.13 -0.12 -0.11 -0.10 -0.09 -0.08 -0.07 -0.06 -0.05 -0.04 -0.03 -0.02 -0.01 0.00 0.01 0.02 0.03 0.04 0.05 0.06 0.07 0.08 0.09 0.10 0.11 0.12 0.13 0.14 0.15]  f_susp_dzdot_bp=[-0.15 -0.14 -0.13 -0.12 -0.11 -0.10 -0.09 -0.08 -0.07 -0.06 -0.05 -0.04 -0.03 -0.02 -0.01 0.00 0.01 0.02 0.03 0.04 0.05 0.06 0.07 0.08 0.09 0.10 0.11 0.12 0.13 0.14 0.15]  f_susp_fmz=zeros(31,31,61,2,4)  f_susp_geom=zeros(31,61,2,3)  f_susp_strgdelta_bp=[-30,-29,-28,-27,-26,-25,-24,-23,-22,-21,-20,-19,-18,-17,-16,-15,-14,-13,-12,-11,-10,-9,-8,-7,-6,-5,-4,-3,-2,-1,0,1,2,3,4,5,6,7,8,9,10,11,12,13,14,15,16,17,18,19,20,21,22,23,24,25,26,27,28,29,30]
  Steer Rate Adapter : Subsystem
  Steering Adapter : Subsystem
  Terminator{,1..3} (4 alike) : Terminator
  Vehicle Adapter : Subsystem
  Wheel  Adapter : Subsystem
  Wheel1 : InportShadow
  independent Suspensions - MacPherson : vehdynlibsuspension/Independent Suspension - MacPherson  ActiveDampEn=off  NumAxl=1  NumWhlsByAxl=2  StrgEnByAxl=1  AntiSwayEnByAxl=1  WhlNumVec="[1  2]"  AxleNumVec="[1  1]"  SuspTypesByAxle=[1]  SuspImage=suspmacp.png  IdealSuspEn=on  IdealSuspAxles=[1]  Kz=Kz  F0z=F0z(1)  Cz=Cz  Hmax=Hmax  f_act_susp_cz=[10000 10000;10000 10000]  f_act_susp_duty_bpt=[0 1]  f_act_susp_zdot_bpt=[-1 1]  Toe=0  RollStrgSlp=0.  ToeStrgSlp=0.  Caster=0.  CasterHslp=0.  CasterStrgSlp=0.  Camber=-0.5*pi/180*0  CamberHslp=0.  CamberStrgSlp=0.  StrgHgtSlp=0.1432  MappedSuspEn=off  MappedSuspAxles="[1  2]"  f_susp_axl_bp=[1 2]  f_susp_dz_bp=[-0.15 -0.14 -0.13 -0.12 -0.11 -0.10 -0.09 -0.08 -0.07 -0.06 -0.05 -0.04 -0.03 -0.02 -0.01 0.00 0.01 0.02 0.03 0.04 0.05 0.06 0.07 0.08 0.09 0.10 0.11 0.12 0.13 0.14 0.15]  f_susp_dzdot_bp=[-0.15 -0.14 -0.13 -0.12 -0.11 -0.10 -0.09 -0.08 -0.07 -0.06 -0.05 -0.04 -0.03 -0.02 -0.01 0.00 0.01 0.02 0.03 0.04 0.05 0.06 0.07 0.08 0.09 0.10 0.11 0.12 0.13 0.14 0.15]  f_susp_fmz=zeros(31,31,61,2,4)  f_susp_geom=zeros(31,61,2,3)  f_susp_strgdelta_bp=[-30,-29,-28,-27,-26,-25,-24,-23,-22,-21,-20,-19,-18,-17,-16,-15,-14,-13,-12,-11,-10,-9,-8,-7,-6,-5,-4,-3,-2,-1,0,1,2,3,4,5,6,7,8,9,10,11,12,13,14,15,16,17,18,19,20,21,22,23,24,25,26,27,28,29,30]  AntiSwayR=0.2  AntiSwayNtrlAng=0.5236  AntiSwayTrsK=8e+02
  Suspension : Outport  VectorParamsAs1DForOutWhenUnconnected=off
  wires:
  Bus Creator3/1 -> Suspension/1
  Bus Creator1/1 -> Bus Creator3/2  "Whl"
  Bus Selector1/2 -> Selector11/1, Selector18/1  "<V>"
  Bus Selector/6 -> Selector9/1, Selector17/1  "<M>"
  Bus Selector/5 -> Selector8/1, Selector16/1  "<Fy>"
  Bus Selector/1 -> Selector3/1, Selector5/1  "<z>"
  Steering/1 -> Steering Adapter/1(Steer)
  Bus Selector1/1 -> Selector10/1, Selector1/1  "<P>"
  Matrix Concatenate/1 -> Bus Creator1/3  "ydot"
  independent Suspensions - MacPherson/6 -> Matrix Concatenate2/1
  Selector12/1 -> Matrix Concatenate1/1
  independent Suspensions - MacPherson/4 -> Matrix Concatenate4/1
  independent Suspensions - MacPherson/1 -> Terminator/1
  Bus Selector/4 -> Selector7/1, Selector21/1  "<Fx>"
  Vehicle Adapter/1(VehSusp) -> Bus Selector1/1
  independent Suspensions - MacPherson/2 -> Matrix Concatenate6/1
  independent Suspensions - MacPherson/3 -> Matrix Concatenate5/1
  Bus Creator2/1 -> Bus Creator3/1  "Veh"
  Steering Adapter/1(StrgAng) -> Selector2/1
  Bus Creator4/1 -> Bus Selector/1
  Wheel  Adapter/2(WhlFy) -> Bus Creator4/2  "Fy"
  Wheel  Adapter/1(WhlFx) -> Bus Creator4/1  "Fx"
  Wheel/1 -> Wheel  Adapter/1(Wheels)
  Wheel  Adapter/3(z) -> Bus Creator4/3
  Wheel  Adapter/4(zdot) -> Bus Creator4/4
  Wheel  Adapter/5(M) -> Bus Creator4/5
  Bus Selector/2 -> Selector20/1, Selector4/1  "<RL>"
  Selector2/1 -> independent Suspensions - MacPherson/9
  Selector3/1 -> Solid Axle Suspension - Coil Spring/1
  Selector4/1 -> independent Suspensions - MacPherson/2
  Selector5/1 -> independent Suspensions - MacPherson/1
  Selector6/1 -> independent Suspensions - MacPherson/3
  Selector7/1 -> independent Suspensions - MacPherson/4
  Selector8/1 -> independent Suspensions - MacPherson/5
  Selector9/1 -> independent Suspensions - MacPherson/6
  Selector10/1 -> independent Suspensions - MacPherson/7
  Selector11/1 -> independent Suspensions - MacPherson/8
  Selector13/1 -> Matrix Concatenate/1
  Selector15/1 -> Matrix Concatenate/2
  Matrix Concatenate1/1 -> Bus Creator1/2  "xdot"
  Selector14/1 -> Matrix Concatenate1/2
  Matrix Concatenate2/1 -> Bus Creator1/4  "Ang"
  Solid Axle Suspension - Coil Spring/6 -> Matrix Concatenate2/2
  Matrix Concatenate4/1 -> Bus Creator1/1  "F"
  Solid Axle Suspension - Coil Spring/4 -> Matrix Concatenate4/2
  Matrix Concatenate5/1 -> Bus Creator2/2  "M"
  Matrix Concatenate6/1 -> Bus Creator2/1  "F"
  Solid Axle Suspension - Coil Spring/2 -> Matrix Concatenate6/2
  Selector16/1 -> Solid Axle Suspension - Coil Spring/5
  Selector17/1 -> Solid Axle Suspension - Coil Spring/6
  Selector1/1 -> Solid Axle Suspension - Coil Spring/7
  Selector18/1 -> Solid Axle Suspension - Coil Spring/8
  Selector20/1 -> Solid Axle Suspension - Coil Spring/2
  Wheel  Adapter/6(RL) -> Bus Creator4/6
  Selector21/1 -> Solid Axle Suspension - Coil Spring/4
  Solid Axle Suspension - Coil Spring/3 -> Matrix Concatenate5/2
  Vehicle/1 -> Vehicle Adapter/1(Veh), Steer Rate Adapter/1(Veh)
  Selector22/1 -> Solid Axle Suspension - Coil Spring/3
  Bus Selector/3 -> Selector22/1, Selector6/1  "<zdot>"
  Solid Axle Suspension - Coil Spring/1 -> Terminator1/1  "Susp"
  Vehicle Adapter/2(VehVbody) -> Selector23/1, Selector19/1
  Steer Rate Adapter/1(AngVel) -> Bus Creator1/6
  independent Suspensions - MacPherson/5 -> Terminator2/1
  Solid Axle Suspension - Coil Spring/5 -> Terminator3/1
  Selector19/1 -> Selector12/1, Selector13/1
  Selector23/1 -> Selector15/1, Selector14/1
  Wheel1/1 -> Bus Selector2/1
  Bus Selector2/1 -> Bus Creator1/5  "<z>"

== system PassVeh14DOF/Suspension/MacPherson Suspension ==
  Wheel : Inport
  Steering : Inport  Port=2
  Vehicle : Inport  Port=3
  Bus Creator1 : BusCreator  Inputs=6
  Bus Creator2 : BusCreator  Inputs=2
  Bus Creator3 : BusCreator  Inputs=2
  Bus Creator4 : BusCreator  Inputs=6
  Bus Selector : BusSelector  OutputSignals=z,RL,zdot,Fx,Fy,M
  Bus Selector1 : BusSelector  OutputSignals=P,V
  Bus Selector2 : BusSelector  OutputSignals=SuspFrame.z
  Selector1 : Selector  NumberOfDimensions=2  IndexOptions=Index vector (dialog),Select all  Indices=1,1  OutputSizes=1,1
  Selector2 : Selector  NumberOfDimensions=2  IndexOptions=Index vector (dialog),Select all  Indices=2,1  OutputSizes=1,1
  Steer Rate Adapter : Subsystem
  Steering Adapter : Subsystem
  Terminator : Terminator
  Terminator1 : Terminator
  Vehicle Adapter : Subsystem
  Wheel  Adapter : Subsystem
  Wheel1 : InportShadow
  independent Suspensions - MacPherson : vehdynlibsuspension/Independent Suspension - MacPherson  ActiveDampEn=off  NumAxl=2  NumWhlsByAxl=[2 2]  StrgEnByAxl=[1 0]  AntiSwayEnByAxl=[1 0]  WhlNumVec="[1  2  1  2]"  AxleNumVec="[1  1  2  2]"  SuspTypesByAxle="[1  1]"  SuspImage=suspmacp.png  IdealSuspEn=on  IdealSuspAxles="[1  2]"  Kz=Kz  F0z=F0z  Cz=Cz  Hmax=Hmax  f_act_susp_cz=[10000 10000;10000 10000]  f_act_susp_duty_bpt=[0 1]  f_act_susp_zdot_bpt=[-1 1]  Toe=0.  RollStrgSlp=0.  ToeStrgSlp=0.  Caster=0.  CasterHslp=0.  CasterStrgSlp=0.  Camber=0.  CamberHslp=0.  CamberStrgSlp=0.  StrgHgtSlp=0.1432  MappedSuspEn=off  MappedSuspAxles="[1  2]"  f_susp_axl_bp=[1 2]  f_susp_dz_bp=[-0.15 -0.14 -0.13 -0.12 -0.11 -0.10 -0.09 -0.08 -0.07 -0.06 -0.05 -0.04 -0.03 -0.02 -0.01 0.00 0.01 0.02 0.03 0.04 0.05 0.06 0.07 0.08 0.09 0.10 0.11 0.12 0.13 0.14 0.15]  f_susp_dzdot_bp=[-0.15 -0.14 -0.13 -0.12 -0.11 -0.10 -0.09 -0.08 -0.07 -0.06 -0.05 -0.04 -0.03 -0.02 -0.01 0.00 0.01 0.02 0.03 0.04 0.05 0.06 0.07 0.08 0.09 0.10 0.11 0.12 0.13 0.14 0.15]  f_susp_fmz=zeros(31,31,61,2,4)  f_susp_geom=zeros(31,61,2,3)  f_susp_strgdelta_bp=[-30,-29,-28,-27,-26,-25,-24,-23,-22,-21,-20,-19,-18,-17,-16,-15,-14,-13,-12,-11,-10,-9,-8,-7,-6,-5,-4,-3,-2,-1,0,1,2,3,4,5,6,7,8,9,10,11,12,13,14,15,16,17,18,19,20,21,22,23,24,25,26,27,28,29,30]  AntiSwayR=0.2  AntiSwayNtrlAng=0.5236  AntiSwayTrsK=8e+02
  Suspension : Outport  VectorParamsAs1DForOutWhenUnconnected=off
  wires:
  Bus Creator3/1 -> Suspension/1
  Bus Creator1/1 -> Bus Creator3/2  "Whl"
  Bus Selector1/2 -> independent Suspensions - MacPherson/8  "<V>"
  Bus Selector/6 -> independent Suspensions - MacPherson/6  "<M>"
  Bus Selector/5 -> independent Suspensions - MacPherson/5  "<Fy>"
  Steering/1 -> Steering Adapter/1(Steer)
  Bus Selector/3 -> independent Suspensions - MacPherson/3  "<zdot>"
  Bus Selector/4 -> independent Suspensions - MacPherson/4  "<Fx>"
  Vehicle/1 -> Vehicle Adapter/1(Veh), Steer Rate Adapter/1(Veh)
  Vehicle Adapter/1(VehSusp) -> Bus Selector1/1
  independent Suspensions - MacPherson/3 -> Bus Creator2/2  "M"
  Wheel  Adapter/2(WhlFy) -> Bus Creator4/2  "Fy"
  Wheel  Adapter/1(WhlFx) -> Bus Creator4/1  "Fx"
  Wheel/1 -> Wheel  Adapter/1(Wheels)
  Wheel  Adapter/3(z) -> Bus Creator4/3
  Wheel  Adapter/4(zdot) -> Bus Creator4/4
  Wheel  Adapter/5(M) -> Bus Creator4/5  "M"
  Wheel  Adapter/6(RL) -> Bus Creator4/6
  Bus Selector/2 -> independent Suspensions - MacPherson/2  "<RL>"
  Selector1/1 -> Bus Creator1/2  "xdot"
  Selector2/1 -> Bus Creator1/3  "ydot"
  Bus Selector1/1 -> independent Suspensions - MacPherson/7  "<P>"
  Bus Selector/1 -> independent Suspensions - MacPherson/1  "<z>"
  independent Suspensions - MacPherson/4 -> Bus Creator1/1  "F"
  independent Suspensions - MacPherson/6 -> Bus Creator1/4  "Ang"
  Vehicle Adapter/2(VehVbody) -> Selector1/1, Selector2/1  "V"
  independent Suspensions - MacPherson/2 -> Bus Creator2/1  "F"
  Bus Creator2/1 -> Bus Creator3/1  "Veh"
  Bus Creator4/1 -> Bus Selector/1
  Steer Rate Adapter/1(AngVel) -> Bus Creator1/6  "AngVel"
  Steering Adapter/1(StrgAng) -> independent Suspensions - MacPherson/9
  independent Suspensions - MacPherson/1 -> Terminator/1
  independent Suspensions - MacPherson/5 -> Terminator1/1  "V"
  Bus Selector2/1 -> Bus Creator1/5  "<z>"
  Wheel1/1 -> Bus Selector2/1

== system PassVeh14DOF/Suspension/Mapped Suspension ==
  Wheel : Inport
  Steering : Inport  Port=2
  Vehicle : Inport  Port=3
  Bus Creator1 : BusCreator  Inputs=6
  Bus Creator2 : BusCreator  Inputs=2
  Bus Creator3 : BusCreator  Inputs=2
  Bus Creator4 : BusCreator  Inputs=6
  Bus Selector : BusSelector  OutputSignals=z,RL,zdot,Fx,Fy,M
  Bus Selector1 : BusSelector  OutputSignals=P,V
  Bus Selector2 : BusSelector  OutputSignals=SuspFrame.z
  Independent Suspension - Mapped : vehdynlibsuspension/Independent Suspension - Mapped  NumAxl=2  NumWhlsByAxl=[2 2]  StrgEnByAxl=[1 0]  AntiSwayEnByAxl=[1 0]  WhlNumVec="[1  2  1  2]"  AxleNumVec="[1  1  2  2]"  SuspTypesByAxle="[2  2]"  SuspImage=suspindmap.png  IdealSuspEn=off  IdealSuspAxles="[1  2]"  Kz=64370  F0z=9810  Cz=10000  Hmax=0.5  Toe=2  RollStrgSlp=-13  ToeStrgSlp=0.01  Caster=4  CasterHslp=-13  CasterStrgSlp=0.01  Camber=4  CamberHslp=-13  CamberStrgSlp=0.01  StrgHgtSlp=0.0025  MappedSuspEn=on  MappedSuspAxles="[1  2]"  f_susp_axl_bp=[1 2]  f_susp_dz_bp=f_susp_dz_bp  f_susp_dzdot_bp=f_susp_dzdot_bp  f_susp_fmz=f_susp_fmz  f_susp_geom=f_susp_geom  f_susp_strgdelta_bp=f_susp_strgdelta_bp  NDFLookupOutType=1:4  NDGLookupOutType=1:3  AntiSwayR=0.2  AntiSwayNtrlAng=0.5236  AntiSwayTrsK=8e2
  Reshape1 : Reshape  OutputDimensionality=Row vector (2-D)
  Selector : Selector  IndexOptions=Index vector (dialog)  Indices=[1 2]  OutputSizes=1
  Selector1 : Selector  NumberOfDimensions=2  IndexOptions=Index vector (dialog),Select all  Indices=1,1  OutputSizes=1,1
  Selector2 : Selector  NumberOfDimensions=2  IndexOptions=Index vector (dialog),Select all  Indices=2,1  OutputSizes=1,1
  Steer Rate Adapter : Subsystem
  Terminator : Terminator
  Terminator1 : Terminator
  Vehicle Adapter : Subsystem
  Wheel  Adapter : Subsystem
  Wheel1 : InportShadow
  Suspension : Outport  VectorParamsAs1DForOutWhenUnconnected=off
  wires:
  Independent Suspension - Mapped/1 -> Terminator/1
  Reshape1/1 -> Independent Suspension - Mapped/9
  Bus Selector/5 -> Independent Suspension - Mapped/5  "<Fy>"
  Bus Selector/2 -> Independent Suspension - Mapped/2  "<RL>"
  Bus Selector1/2 -> Independent Suspension - Mapped/8  "<V>"
  Bus Selector/4 -> Independent Suspension - Mapped/4  "<Fx>"
  Wheel  Adapter/5(M) -> Bus Creator4/5
  Bus Selector/6 -> Independent Suspension - Mapped/6  "<M>"
  Wheel  Adapter/4(zdot) -> Bus Creator4/4
  Wheel  Adapter/6(RL) -> Bus Creator4/6
  Selector/1 -> Reshape1/1
  Bus Creator4/1 -> Bus Selector/1
  Wheel  Adapter/3(z) -> Bus Creator4/3
  Wheel  Adapter/2(WhlFy) -> Bus Creator4/2  "Fy"
  Wheel/1 -> Wheel  Adapter/1(Wheels)
  Vehicle Adapter/1(VehSusp) -> Bus Selector1/1
  Bus Selector/3 -> Independent Suspension - Mapped/3  "<zdot>"
  Bus Selector/1 -> Independent Suspension - Mapped/1  "<z>"
  Wheel  Adapter/1(WhlFx) -> Bus Creator4/1  "Fx"
  Bus Selector1/1 -> Independent Suspension - Mapped/7  "<P>"
  Steering/1 -> Selector/1
  Vehicle/1 -> Vehicle Adapter/1(Veh), Steer Rate Adapter/1(Veh)
  Independent Suspension - Mapped/6 -> Bus Creator1/4  "Ang"
  Selector2/1 -> Bus Creator1/3  "ydot"
  Independent Suspension - Mapped/2 -> Bus Creator2/1  "F"
  Independent Suspension - Mapped/3 -> Bus Creator2/2  "M"
  Bus Creator2/1 -> Bus Creator3/1  "Veh"
  Bus Creator1/1 -> Bus Creator3/2  "Whl"
  Independent Suspension - Mapped/4 -> Bus Creator1/1  "F"
  Selector1/1 -> Bus Creator1/2  "xdot"
  Vehicle Adapter/2(VehVbody) -> Selector1/1, Selector2/1  "V"
  Bus Creator3/1 -> Suspension/1
  Steer Rate Adapter/1(AngVel) -> Bus Creator1/6
  Independent Suspension - Mapped/5 -> Terminator1/1  "V"
  Bus Selector2/1 -> Bus Creator1/5  "<z>"
  Wheel1/1 -> Bus Selector2/1

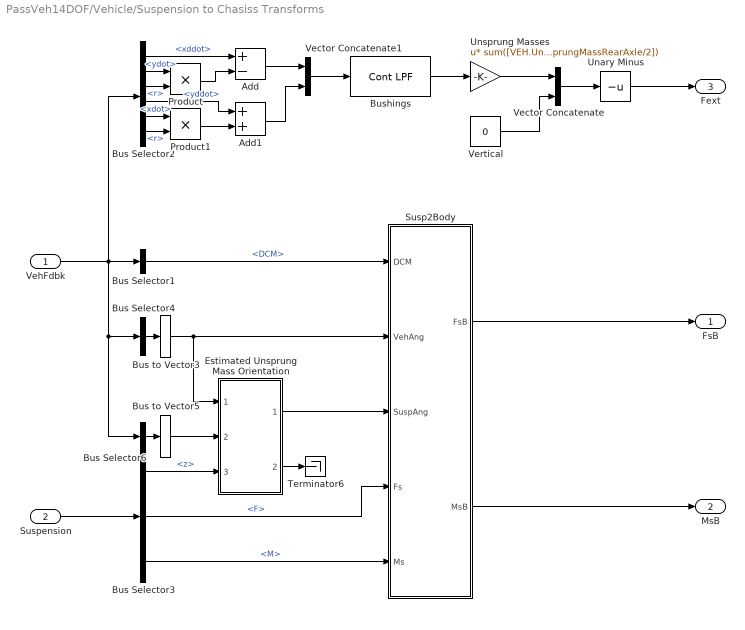
== system PassVeh14DOF/Vehicle/Suspension to Chasiss Transforms ==
  VehFdbk : Inport
  Suspension : Inport  Port=2
  Add : Sum  Inputs=+-
  Add1 : Sum
  Bus Selector1 : BusSelector  OutputSignals=BdyFrm.Cg.DCM
  Bus Selector2 : BusSelector  OutputSignals=BdyFrm.Cg.Acc.xddot,BdyFrm.Cg.Vel.ydot,BdyFrm.Cg.AngVel.r,BdyFrm.Cg.Acc.yddot,BdyFrm.Cg.Vel.xdot,BdyFrm.Cg.AngVel.r
  Bus Selector3 : BusSelector  OutputSignals=Whl.z,Veh.F,Veh.M
  Bus Selector4 : BusSelector  OutputSignals=InertFrm.Cg.Ang.phi,InertFrm.Cg.Ang.theta,InertFrm.Cg.Ang.psi  OutputAsBus=on
  Bus Selector6 : BusSelector  OutputSignals=InertFrm.Geom.Disp.X,InertFrm.Geom.Disp.Y,InertFrm.Geom.Disp.Z  OutputAsBus=on
  Bus to Vector3 : BusToVector
  Bus to Vector5 : BusToVector
  Bushings : autolibutils/Cont LPF  wc=40*pi  AbsoluteTolerance=auto  aMode=2
  Estimated Unsprung Mass Orientation : MATLAB Function  TreatAsAtomicUnit=on  mask{trackW=VEH.TrackWidth, wheelB=VEH.FrontAxlePositionfromCG+VEH.RearAxlePositionfromCG}
      mask prompts: trackW "Vehicle track width, trackW [m]:"; wheelB "Vehicle wheelbase, wheelB [m]:"
      mask help: This block converts wheel ground height information into estimates of vehicle pitch, roll angles and vertical height in order to help in the visualization 3DOF based simulations with changes in terrain. Note that the resulting signals are only used as a visualization aid and do not account for the physical affects of the vehicle interacting with variable terrain or changes in orientation.
  Product : Product
  Product1 : Product
  Susp2Body : Subsystem
  Terminator6 : Terminator
  Unary Minus : UnaryMinus
  Unsprung Masses : Gain  Gain=sum([VEH.UnsprungMassFrontAxle/2 VEH.UnsprungMassFrontAxle/2 VEH.UnsprungMassRearAxle/2 VEH.UnsprungMassRearAxle/2])  Multiplication=Matrix(u*K)
  Vector Concatenate : Concatenate
  Vector Concatenate1 : Concatenate
  Vertical : Constant  Value=0
  FsB : Outport
  MsB : Outport  Port=2
  Fext : Outport  Port=3
  wires:
  Bus Selector6/1 -> Bus to Vector5/1
  Bus Selector3/2 -> Susp2Body/4(Fs)  "<F>"
  VehFdbk/1 -> Bus Selector2/1, Bus Selector1/1, Bus Selector6/1, Bus Selector4/1
  Bus Selector3/3 -> Susp2Body/5(Ms)  "<M>"
  Bus to Vector3/1 -> Estimated Unsprung Mass Orientation/1(angleIn), Susp2Body/2(VehAng)
  Bus Selector1/1 -> Susp2Body/1(DCM)  "<DCM>"
  Bus to Vector5/1 -> Estimated Unsprung Mass Orientation/2(GemoXYZIn)
  Suspension/1 -> Bus Selector3/1
  Bus Selector4/1 -> Bus to Vector3/1
  Estimated Unsprung Mass Orientation/2(GeomXYZ) -> Terminator6/1
  Bus Selector3/1 -> Estimated Unsprung Mass Orientation/3(Ground)  "<z>"
  Estimated Unsprung Mass Orientation/1(angles) -> Susp2Body/3(SuspAng)
  Susp2Body/2(MsB) -> MsB/1
  Bushings/1 -> Unsprung Masses/1
  Vector Concatenate1/1 -> Bushings/1
  Unsprung Masses/1 -> Vector Concatenate/1
  Susp2Body/1(FsB) -> FsB/1
  Vector Concatenate/1 -> Unary Minus/1
  Vertical/1 -> Vector Concatenate/2
  Bus Selector2/2 -> Product/1  "<ydot>"
  Bus Selector2/3 -> Product/2  "<r>"
  Bus Selector2/5 -> Product1/1  "<xdot>"
  Bus Selector2/6 -> Product1/2  "<r>"
  Add/1 -> Vector Concatenate1/1
  Product/1 -> Add/2
  Product1/1 -> Add1/2
  Bus Selector2/4 -> Add1/1  "<yddot>"
  Add1/1 -> Vector Concatenate1/2
  Bus Selector2/1 -> Add/1  "<xddot>"
  Unary Minus/1 -> Fext/1
